simulink model "RadarInput"  (R2024a)
settings: Solver=FixedStepDiscrete  StartTime=0.0  StopTime=RIN_Stop_Time  FixedStep=RIN_Step_Size  RelTol=1e-3  EnableMultiTasking=on
undefined symbols (not defined in the file): RADAR_DIST_FAILSAFE_M, RADAR_RAW_MAX, RADAR_RAW_MIN, RADAR_RECOVERY_CNT, RADAR_RESOLUTION_M, RADAR_STATUS_VALID_CODE, RadarStatus_T, RIN_Counter
libraries: simulink x8
settings Model: DataDictionary=bsd.sldd  Creator=pc  LastModifiedBy=pc
settings OptimizationCC: DefaultParameterBehavior=Inlined  UseDivisionForNetSlopeComputation=on  GainParamInheritBuiltInType=on  UseFloatMulNetSlope=on  InheritOutputTypeSmallerThanSingle=on  UseSpecifiedMinMax=on  InlineInvariantSignals=on  EnhancedBackFolding=on  CachingGlobalReferences=on  BitwiseOrLogicalOp=Bitwise operator  ZeroExternalMemoryAtStartup=off  ZeroInternalMemoryAtStartup=off  NoFixptDivByZeroProtection=on  EfficientFloat2IntCast=on  LifeSpan=2  OptimizeBlockOrder=speed  DifferentSizesBufferReuse=on  EfficientTunableParamExpr=on
settings DebuggingCC: SignalInfNanChecking=warning  ReadBeforeWriteMsg=DisableAll  WriteAfterWriteMsg=DisableAll  WriteAfterReadMsg=DisableAll  MultiTaskDSMMsg=none  IntegerOverflowMsg=error  ParameterTunabilityLossMsg=error  AssertControl=DisableAll  SFUndirectedBroadcastEventsDiag=error
settings HardwareCC: ProdLongLongMode=on
settings ModelReferenceCC: UpdateModelReferenceTargets=IfOutOfDate
settings SFSimCC: CompileTimeRecursionLimit=0  EnableRuntimeRecursion=off  MATLABDynamicMemAlloc=off
settings RTWCC: Description=AUTOSAR  SystemTargetFile=autosar.tlc  GenCodeOnly=on  TemplateMakefile=ert_default_tmf  GenerateReport=on  BuildConfiguration=Faster Runs  IncludeHyperlinkInReport=on  LaunchReport=on  DataTypeReplacement=CDataTypesFixedWidth  GenerateTraceInfo=on  GenerateTraceReport=on  GenerateTraceReportSl=on  GenerateTraceReportSf=on  GenerateTraceReportEml=on
settings CodeAppCC: ForceParamTrailComments=on  IgnoreCustomStorageClasses=off  OperatorAnnotations=on  SimulinkDataObjDesc=on  SFDataObjDesc=on  MATLABFcnDesc=on  InsertBlockDesc=on  StateflowObjectComments=on  MATLABSourceComments=on  EnableCustomComments=on  ReqsInCode=on
settings STFCustomTargetCC: UtilityFuncGeneration=Shared location  MultiwordLength=256  ParMdlRefBuildCompliant=on  CompOptLevelCompliant=on  IncludeMdlTerminateFcn=off  CombineOutputUpdateFcns=on  CombineSignalStateStructs=on  SuppressErrorStatus=on  ERTCustomFileBanners=on  SupportNonFinite=off  SupportComplex=off  SupportContinuousTime=off  SupportNonInlinedSFcns=off  RemoveResetFunc=on  ParenthesesLevel=Standards  CastingMode=Standards  MATLABClassNameForMDSCustomization=Simulink.SoftwareTarget.ERTCustomization  AutosarCompliant=on  GRTInterface=off  GenerateSharedConstants=off  LookupTableObjectStructAxisOrder=2,1,3,4,...  LUTObjectStructOrderEvenSpacing=Size,Table,Breakpoints  SystemTargetFile=autosar.tlc
settings ERTTargetCC: TargetLangStandard=C99 (ISO)  UtilityFuncGeneration=Shared location  ConcurrentExecutionCompliant=off  IncludeMdlTerminateFcn=off  CombineSignalStateStructs=on  SuppressErrorStatus=on  SupportNonFinite=off  SupportComplex=off  ParenthesesLevel=Standards  CastingMode=Standards  ModelStepFunctionPrototypeControlCompliant=off  CPPClassGenCompliant=off  AutosarCompliant=on  GenerateSharedConstants=off  LookupTableObjectStructAxisOrder=2,1,3,4,...  LUTObjectStructOrderEvenSpacing=Size,Table,Breakpoints  InlinedParameterPlacement=NonHierarchical  ERTCustomFileTemplate=example_file_process.tlc  EnableSignedLeftShifts=off  EnableSignedRightShifts=off  BooleanTrueId=TRUE  BooleanFalseId=FALSE

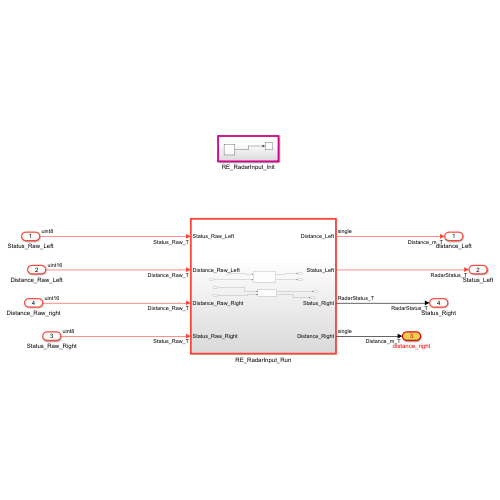
[thumbnail: Simulink's stored preview of the top-level diagram]
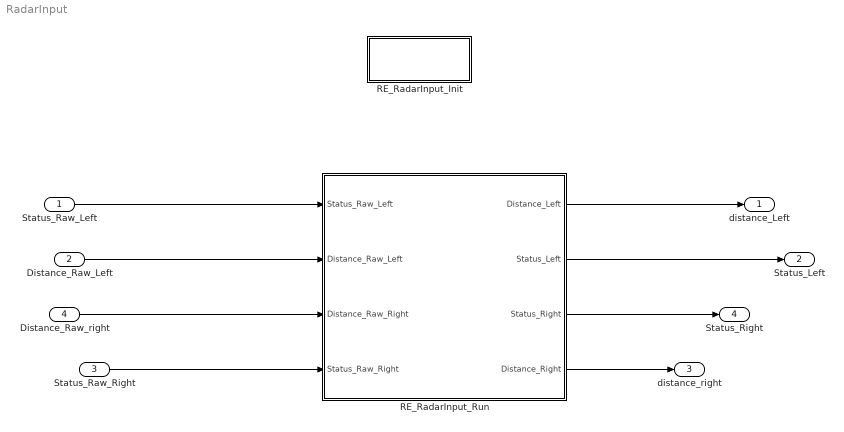
== system RadarInput ==
  Status_Raw_Left : Inport  OutDataTypeStr=Status_Raw_T
  Distance_Raw_Left : Inport  Port=2  OutDataTypeStr=Distance_Raw_T
  Status_Raw_Right : Inport  Port=3  OutDataTypeStr=Status_Raw_T
  Distance_Raw_right : Inport  Port=4  OutDataTypeStr=Distance_Raw_T
  RE_RadarInput_Init : Subsystem  TreatAsAtomicUnit=on
  RE_RadarInput_Run : Subsystem  TreatAsAtomicUnit=on
  distance_Left : Outport  OutDataTypeStr=Distance_m_T
  Status_Left : Outport  Port=2  OutDataTypeStr=Enum: RadarStatus_T
  distance_right : Outport  Port=3  OutDataTypeStr=Distance_m_T
  Status_Right : Outport  Port=4  OutDataTypeStr=Enum: RadarStatus_T
  wires:
  RE_RadarInput_Run/2(Status_Left) -> Status_Left/1
  RE_RadarInput_Run/4(Distance_Right) -> distance_right/1
  RE_RadarInput_Run/1(Distance_Left) -> distance_Left/1
  RE_RadarInput_Run/3(Status_Right) -> Status_Right/1
  Status_Raw_Left/1 -> RE_RadarInput_Run/1(Status_Raw_Left)
  Distance_Raw_Left/1 -> RE_RadarInput_Run/2(Distance_Raw_Left)
  Distance_Raw_right/1 -> RE_RadarInput_Run/3(Distance_Raw_Right)
  Status_Raw_Right/1 -> RE_RadarInput_Run/4(Status_Raw_Right)

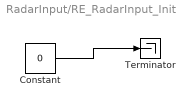
== system RadarInput/RE_RadarInput_Init ==
  Constant : Constant  Value=0
  Terminator : Terminator
  wires:
  Constant/1 -> Terminator/1

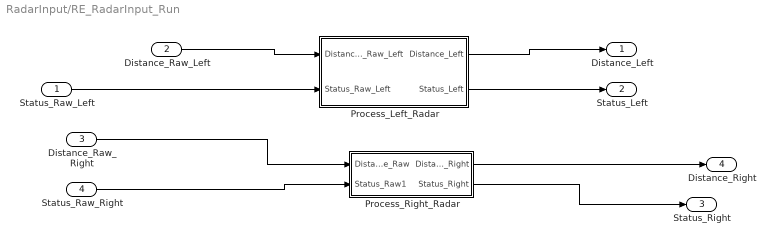
== system RadarInput/RE_RadarInput_Run ==
  Status_Raw_Left : Inport  OutDataTypeStr=Status_Raw_T
  Distance_Raw_Left : Inport  Port=2  OutDataTypeStr=Distance_Raw_T
  Distance_Raw_Right : Inport  Port=3  OutDataTypeStr=Distance_Raw_T
  Status_Raw_Right : Inport  Port=4  OutDataTypeStr=Status_Raw_T
  Process_Left_Radar : Subsystem
  Process_Right_Radar : Subsystem
  Distance_Left : Outport  OutDataTypeStr=Distance_m_T
  Status_Left : Outport  Port=2
  Status_Right : Outport  Port=3  OutDataTypeStr=Enum: RadarStatus_T
  Distance_Right : Outport  Port=4  OutDataTypeStr=Distance_m_T
  wires:
  Process_Left_Radar/1(Distance_Left) -> Distance_Left/1
  Process_Right_Radar/1(Distance_Right) -> Distance_Right/1
  Process_Left_Radar/2(Status_Left) -> Status_Left/1
  Distance_Raw_Right/1 -> Process_Right_Radar/1(Distance_Raw)
  Process_Right_Radar/2(Status_Right) -> Status_Right/1
  Status_Raw_Right/1 -> Process_Right_Radar/2(Status_Raw1)
  Distance_Raw_Left/1 -> Process_Left_Radar/1(Distance_Raw_Left)
  Status_Raw_Left/1 -> Process_Left_Radar/2(Status_Raw_Left)

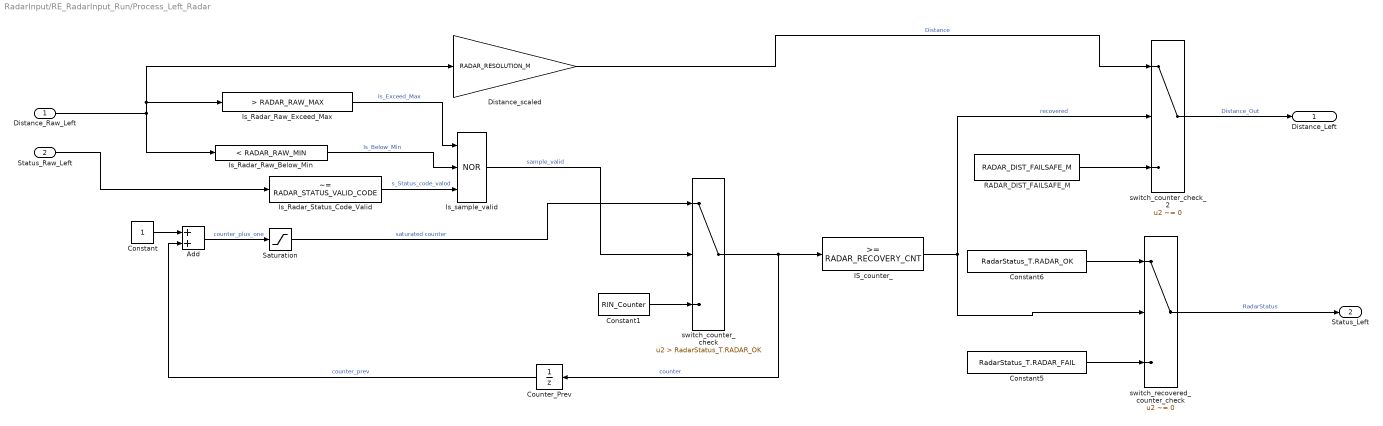
== system RadarInput/RE_RadarInput_Run/Process_Left_Radar ==
  Distance_Raw_Left : Inport  OutDataTypeStr=Distance_Raw_T
  Status_Raw_Left : Inport  Port=2  OutDataTypeStr=Status_Raw_T
  Add : Sum  OutDataTypeStr=uint8
  Constant : Constant  OutDataTypeStr=uint8
  Constant1 : Constant  Value=RIN_Counter
  Constant5 : Constant  Value=RadarStatus_T.RADAR_FAIL  OutDataTypeStr=Enum: RadarStatus_T
  Constant6 : Constant  Value=RadarStatus_T.RADAR_OK  OutDataTypeStr=Enum: RadarStatus_T
  Counter_Prev : UnitDelay  SampleTime=-1  HasFrameUpgradeWarning=on
  Distance_scaled : Gain  Gain=RADAR_RESOLUTION_M  ParamDataTypeStr=single  OutDataTypeStr=single
  IS_counter_ : simulink/Logic and Bit Operations/Compare To Constant  relop=>=  const=RADAR_RECOVERY_CNT  OutDataTypeStr=boolean
  Is_Radar_Raw_Below_Min : simulink/Logic and Bit Operations/Compare To Constant  relop=<  const=RADAR_RAW_MIN  OutDataTypeStr=boolean
  Is_Radar_Raw_Exceed_Max : simulink/Logic and Bit Operations/Compare To Constant  relop=>  const=RADAR_RAW_MAX  OutDataTypeStr=boolean
  Is_Radar_Status_Code_Valid : simulink/Logic and Bit Operations/Compare To Constant  relop=~=  const=RADAR_STATUS_VALID_CODE  OutDataTypeStr=boolean
  Is_sample_valid : Logic  Operator=NOR  Inputs=3  AllPortsSameDT=off  OutDataTypeStr=boolean
  RADAR_DIST_FAILSAFE_M : Constant  Value=RADAR_DIST_FAILSAFE_M  OutDataTypeStr=ValueType: Distance
  Saturation : Saturate  UpperLimit=RADAR_RECOVERY_CNT  LowerLimit=0  OutDataTypeStr=uint8
  switch_counter_check : Switch  Criteria=u2 > Threshold  Threshold=RadarStatus_T.RADAR_OK  OutDataTypeStr=uint8  SaturateOnIntegerOverflow=off  InputSameDT=off
  switch_counter_check_2 : Switch  Criteria=u2 ~= 0  OutDataTypeStr=single  SaturateOnIntegerOverflow=off  InputSameDT=off
  switch_recovered_counter_check : Switch  Criteria=u2 ~= 0  OutDataTypeStr=Enum: RadarStatus_T  SaturateOnIntegerOverflow=off  InputSameDT=off
  Distance_Left : Outport  OutDataTypeStr=Distance_m_T
  Status_Left : Outport  Port=2  OutDataTypeStr=Enum: RadarStatus_T
  wires:
  Distance_scaled/1 -> switch_counter_check_2/1  "Distance"
  Constant6/1 -> switch_recovered_counter_check/1
  switch_recovered_counter_check/1 -> Status_Left/1  "RadarStatus"
  Distance_Raw_Left/1 -> Distance_scaled/1, Is_Radar_Raw_Exceed_Max/1, Is_Radar_Raw_Below_Min/1
  Status_Raw_Left/1 -> Is_Radar_Status_Code_Valid/1
  Is_Radar_Status_Code_Valid/1 -> Is_sample_valid/3  "s_Status_code_valod"
  Is_sample_valid/1 -> switch_counter_check/2  "sample_valid"
  Is_Radar_Raw_Below_Min/1 -> Is_sample_valid/2  "Is_Below_Min"
  Is_Radar_Raw_Exceed_Max/1 -> Is_sample_valid/1  "Is_Exceed_Max"
  Constant/1 -> Add/1
  Saturation/1 -> switch_counter_check/1  "saturated counter"
  Counter_Prev/1 -> Add/2  "counter_prev"
  Add/1 -> Saturation/1  "counter_plus_one"
  Constant1/1 -> switch_counter_check/3
  switch_counter_check/1 -> Counter_Prev/1, IS_counter_/1  "counter"
  IS_counter_/1 -> switch_recovered_counter_check/2, switch_counter_check_2/2  "recovered"
  Constant5/1 -> switch_recovered_counter_check/3
  switch_counter_check_2/1 -> Distance_Left/1  "Distance_Out"
  RADAR_DIST_FAILSAFE_M/1 -> switch_counter_check_2/3

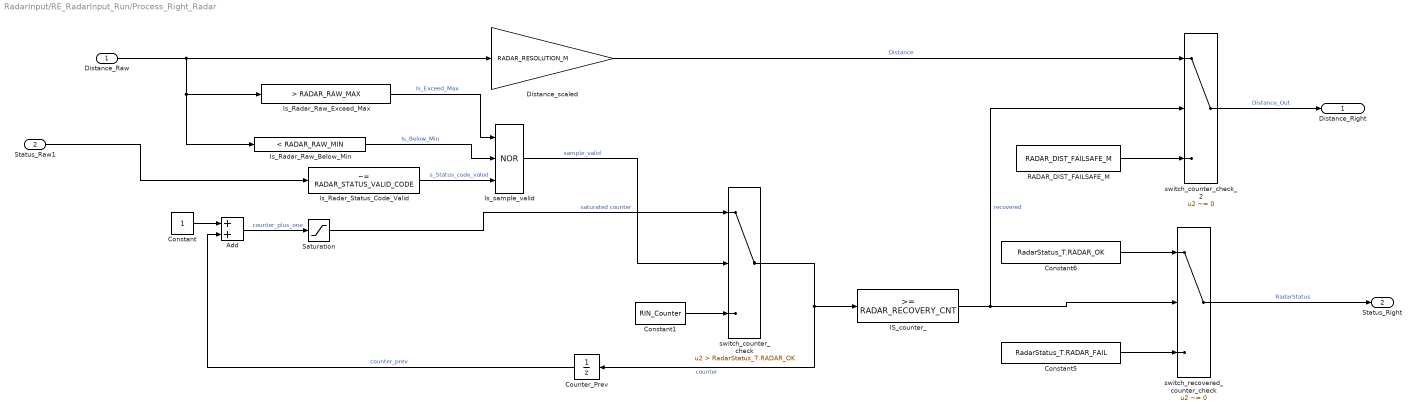
== system RadarInput/RE_RadarInput_Run/Process_Right_Radar ==
  Distance_Raw : Inport  OutDataTypeStr=Distance_Raw_T
  Status_Raw1 : Inport  Port=2  OutDataTypeStr=Status_Raw_T
  Add : Sum  OutDataTypeStr=uint8
  Constant : Constant  OutDataTypeStr=uint8
  Constant1 : Constant  Value=RIN_Counter
  Constant5 : Constant  Value=RadarStatus_T.RADAR_FAIL  OutDataTypeStr=Enum: RadarStatus_T
  Constant6 : Constant  Value=RadarStatus_T.RADAR_OK  OutDataTypeStr=Enum: RadarStatus_T
  Counter_Prev : UnitDelay  SampleTime=-1  HasFrameUpgradeWarning=on
  Distance_scaled : Gain  Gain=RADAR_RESOLUTION_M  ParamDataTypeStr=single  OutDataTypeStr=single
  IS_counter_ : simulink/Logic and Bit Operations/Compare To Constant  relop=>=  const=RADAR_RECOVERY_CNT  OutDataTypeStr=boolean
  Is_Radar_Raw_Below_Min : simulink/Logic and Bit Operations/Compare To Constant  relop=<  const=RADAR_RAW_MIN  OutDataTypeStr=boolean
  Is_Radar_Raw_Exceed_Max : simulink/Logic and Bit Operations/Compare To Constant  relop=>  const=RADAR_RAW_MAX  OutDataTypeStr=boolean
  Is_Radar_Status_Code_Valid : simulink/Logic and Bit Operations/Compare To Constant  relop=~=  const=RADAR_STATUS_VALID_CODE  OutDataTypeStr=boolean
  Is_sample_valid : Logic  Operator=NOR  Inputs=3  AllPortsSameDT=off  OutDataTypeStr=boolean
  RADAR_DIST_FAILSAFE_M : Constant  Value=RADAR_DIST_FAILSAFE_M  OutDataTypeStr=ValueType: Distance
  Saturation : Saturate  UpperLimit=RADAR_RECOVERY_CNT  LowerLimit=0  OutDataTypeStr=uint8
  switch_counter_check : Switch  Criteria=u2 > Threshold  Threshold=RadarStatus_T.RADAR_OK  OutDataTypeStr=uint8  SaturateOnIntegerOverflow=off  InputSameDT=off
  switch_counter_check_2 : Switch  Criteria=u2 ~= 0  OutDataTypeStr=single  SaturateOnIntegerOverflow=off  InputSameDT=off
  switch_recovered_counter_check : Switch  Criteria=u2 ~= 0  OutDataTypeStr=Enum: RadarStatus_T  SaturateOnIntegerOverflow=off  InputSameDT=off
  Distance_Right : Outport  OutDataTypeStr=Distance_m_T
  Status_Right : Outport  Port=2  OutDataTypeStr=Enum: RadarStatus_T
  wires:
  Saturation/1 -> switch_counter_check/1  "saturated counter"
  Constant1/1 -> switch_counter_check/3
  Add/1 -> Saturation/1  "counter_plus_one"
  switch_counter_check_2/1 -> Distance_Right/1  "Distance_Out"
  Is_Radar_Status_Code_Valid/1 -> Is_sample_valid/3  "s_Status_code_valod"
  Distance_scaled/1 -> switch_counter_check_2/1  "Distance"
  Constant6/1 -> switch_recovered_counter_check/1
  IS_counter_/1 -> switch_counter_check_2/2, switch_recovered_counter_check/2  "recovered"
  Constant/1 -> Add/1
  Constant5/1 -> switch_recovered_counter_check/3
  Status_Raw1/1 -> Is_Radar_Status_Code_Valid/1
  switch_counter_check/1 -> Counter_Prev/1, IS_counter_/1  "counter"
  Is_sample_valid/1 -> switch_counter_check/2  "sample_valid"
  Is_Radar_Raw_Exceed_Max/1 -> Is_sample_valid/1  "Is_Exceed_Max"
  switch_recovered_counter_check/1 -> Status_Right/1  "RadarStatus"
  Is_Radar_Raw_Below_Min/1 -> Is_sample_valid/2  "Is_Below_Min"
  Counter_Prev/1 -> Add/2  "counter_prev"
  Distance_Raw/1 -> Is_Radar_Raw_Below_Min/1, Is_Radar_Raw_Exceed_Max/1, Distance_scaled/1
  RADAR_DIST_FAILSAFE_M/1 -> switch_counter_check_2/3
